simulink model "SEA_LQG_nonlinear"  (R2025b)
settings: Solver=ode23t  StartTime=0.0  StopTime=4  MaxStep=0.0050000000000000001  RelTol=1.0000000000000001e-05  AbsTol=9.9999999999999995e-08
Description:
  | explicit LQR plus Kalman observer -> M3 actuators -> nonlinear M1 SEA
settings Model: Creator=aless  LastModifiedBy=aless

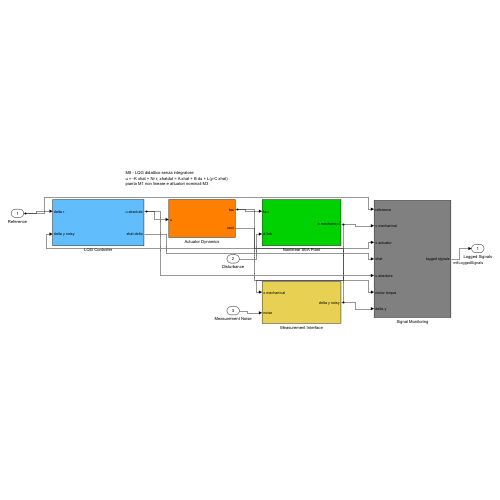
[thumbnail: Simulink's stored preview of the top-level diagram]
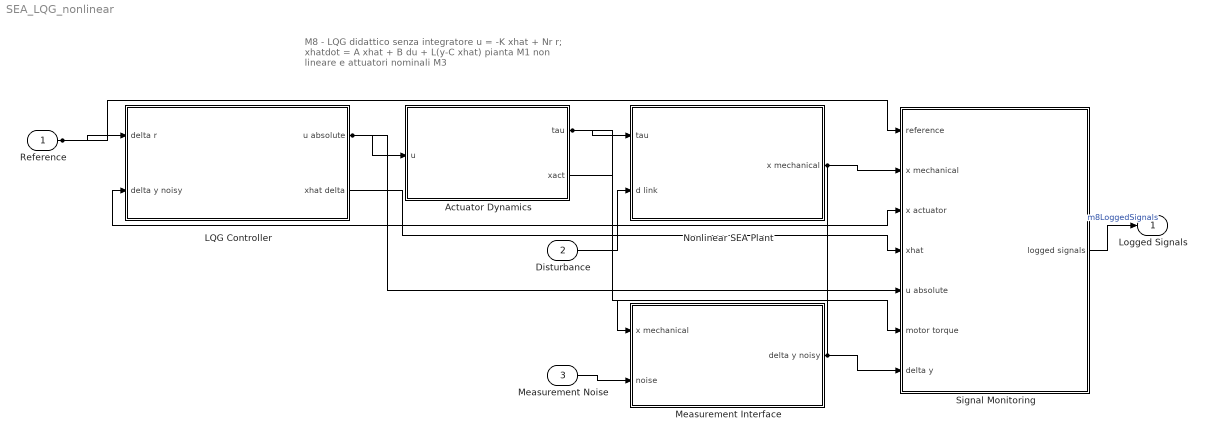
== system SEA_LQG_nonlinear ==
  note: M8 - LQG didattico senza integratore
      | u = -K xhat + Nr r; xhatdot = A xhat + B du + L(y-C xhat)
      | pianta M1 non lineare e attuatori nominali M3
  Reference : Inport  PortDimensions=2
  Disturbance : Inport  Port=2  PortDimensions=2
  Measurement Noise : Inport  Port=3  PortDimensions=4
  Actuator Dynamics : Subsystem
  LQG Controller : Subsystem
  Measurement Interface : Subsystem
  Nonlinear SEA Plant : Subsystem
  Signal Monitoring : Subsystem
  Logged Signals : Outport
  wires:
  Reference/1 -> LQG Controller/1(delta r), Signal Monitoring/1(reference)
  Measurement Interface/1(delta y noisy) -> LQG Controller/2(delta y noisy), Signal Monitoring/7(delta y)
  LQG Controller/1(u absolute) -> Actuator Dynamics/1(u), Signal Monitoring/5(u absolute)
  Actuator Dynamics/1(tau) -> Nonlinear SEA Plant/1(tau), Signal Monitoring/6(motor torque)
  Disturbance/1 -> Nonlinear SEA Plant/2(d link)
  Nonlinear SEA Plant/1(x mechanical) -> Measurement Interface/1(x mechanical), Signal Monitoring/2(x mechanical)
  Measurement Noise/1 -> Measurement Interface/2(noise)
  Actuator Dynamics/2(xact) -> Signal Monitoring/3(x actuator)
  LQG Controller/2(xhat delta) -> Signal Monitoring/4(xhat)
  Signal Monitoring/1(logged signals) -> Logged Signals/1  "m8LoggedSignals"

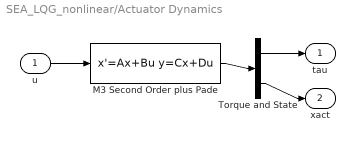
== system SEA_LQG_nonlinear/Actuator Dynamics ==
  u : Inport  PortDimensions=2
  M3 Second Order plus Pade : StateSpace  A=[-197.33333333333334 -79.166666666666671 -52.083333333333336 0 0 0;128 0 0 0 0 0;0 32 0 0 0 0;0 0 0 -197.33333333333334 -79.166666666666671 -52.083333333333336;0 0 0 128 0 0;0 0 0 0 32 0]  B=[8 0;0 0;0 0;0 8;0 0;0 0]  C=[0 -1.5625 6.510416666666667 0 0 0;0 0 0 0 -1.5625 6.510416666666667;1 0 0 0 0 0;0 1 0 0 0 0;0 0 1 0 0 0;0 0 0 1 0 0;0 0 0 0 1 0;0 0 0 0 0 1]  D=[0 0;0 0;0 0;0 0;0 0;0 0;0 0;0 0]  InitialCondition=[0;0;8.8575234782592865e-17;0;0;2.2143808695648216e-17]
  Torque and State : Demux  Outputs=[2 6]
  tau : Outport
  xact : Outport  Port=2
  wires:
  u/1 -> M3 Second Order plus Pade/1
  M3 Second Order plus Pade/1 -> Torque and State/1
  Torque and State/1 -> tau/1
  Torque and State/2 -> xact/1

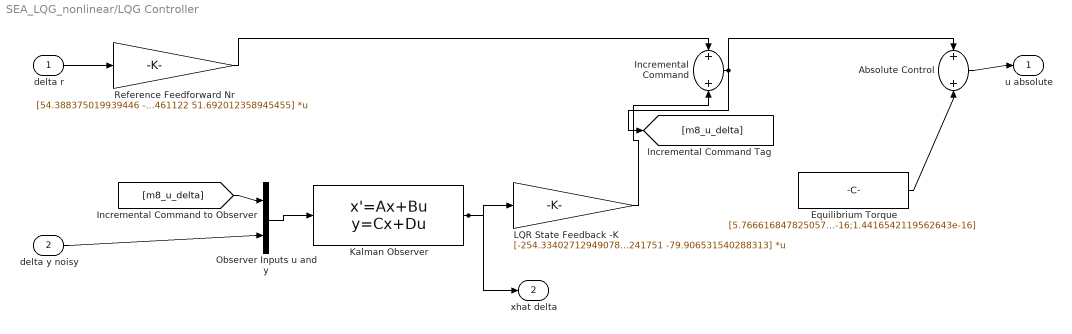
== system SEA_LQG_nonlinear/LQG Controller ==
  delta r : Inport  PortDimensions=2
  delta y noisy : Inport  Port=2  PortDimensions=4
  Absolute Control : Sum
  Equilibrium Torque : Constant  Value=[5.766616847825057e-16;1.4416542119562643e-16]
  Incremental Command : Sum
  Kalman Observer : StateSpace  A=[-22.708602708322911 21.793600911689683 1 0 -9.0440803445696254 5.5226633937677452 0 0 0 0 0 0 0 0;21.793600911690966 -85.604320358251826 0 1 6.9226259293456325 -23.470979906457924 0 0 0 0 0 0 0 0;-839.44343895121312 1838.0863088093163 0 0 79.231545442824768 -233.95675516648708 0 0 0 0 0 0 0 0;1983.0284167279717 -6039.1218427782769 0 0 -347.56991299100787 706.11322932558824 0 0 0 0 0 0 0 0;-9.0440803445693483 6.9226259293442176 0 0 -64.379631998469478 3.421864338890741 1 0 0 0 0 0 0 0;5.5226633937682017 -23.470979906457945 0 0 3.4218643388915506 -79.196108971786572 0 1 0 0 0 0 0 0;4275.8687111143208 934.10363067824846 0 0 -7143.0821554243939 313.4488480155174 -2 0 0 -156.25 651.04166666666674 0 0 0;755.87362777812768 1198.4788631876099 0 0 390.2760854773058 -7432.5597702775658 0 -2 0 0 0 0 -156.25 651.04166666666674;0.41526297627126696 2.254054873951131 0 0 35.114552541148264 1.7286492797991677 0 0 -197.33333333333334 -79.166666666666671 -52.083333333333336 0 0 0;-24.319927449188871 -14.409023934576732 0 0 92.13651423381539 0.28862886679991817 0 0 128 0 0 0 0 0;30.066433915707986 12.673170158948555 0 0 -207.8279927246254 -4.7947871057936995 0 0 0 32 0 0 0 0;1.9578954483030317 -4.8132582922373981 0 0 1.7024879035052436 30.031818202917915 0 0 0 0 0 -197.33333333333334 -79.166666666666671 -52.083333333333336;-11.539925704793928 9.1650966677943853 0 0 -1.3604732519714573 101.985096573353 0 0 0 0 0 128 0 0;9.7588925544826317 0.59061749336000824 0 0 -2.6169632704474655 -207.4223782133657 0 0 0 0 0 0 32 0]  B=[0 0 22.708602708322911 -21.793600911689683 9.0440803445696254 -5.5226633937677452;0 0 -21.793600911690966 85.604320358251826 -6.9226259293456325 23.470979906457924;0 0 551.4684389512131 -1274.3729754759829 233.26845455717523 -349.37657816684629;0 0 -1278.3867500613051 4200.9351761116104 -381.59675367565876 1210.5534373410785;0 0 9.0440803445693483 -6.9226259293442176 64.379631998469478 -3.421864338890741;0 0 -5.5226633937682017 23.470979906457945 -3.4218643388915506 79.196108971786572;0 0 724.13128888567894 -934.10363067824846 2143.0821554243939 -313.4488480155174;0 0 -755.87362777812768 2801.5211368123901 -390.2760854773058 3432.5597702775658;8 0 -0.41526297627126696 -2.254054873951131 -35.114552541148264 -1.7286492797991677;0 0 24.319927449188871 14.409023934576732 -92.13651423381539 -0.28862886679991817;0 0 -30.066433915707986 -12.673170158948555 207.8279927246254 4.7947871057936995;0 8 -1.9578954483030317 4.8132582922373981 -1.7024879035052436 -30.031818202917915;0 0 11.539925704793928 -9.1650966677943853 1.3604732519714573 -101.985096573353;0 0 -9.7588925544826317 -0.59061749336000824 2.6169632704474655 207.4223782133657]  C=[1 0 0 0 0 0 0 0 0 0 0 0 0 0;0 1 0 0 0 0 0 0 0 0 0 0 0 0;0 0 1 0 0 0 0 0 0 0 0 0 0 0;0 0 0 1 0 0 0 0 0 0 0 0 0 0;0 0 0 0 1 0 0 0 0 0 0 0 0 0;0 0 0 0 0 1 0 0 0 0 0 0 0 0;0 0 0 0 0 0 1 0 0 0 0 0 0 0;0 0 0 0 0 0 0 1 0 0 0 0 0 0;0 0 0 0 0 0 0 0 1 0 0 0 0 0;0 0 0 0 0 0 0 0 0 1 0 0 0 0;0 0 0 0 0 0 0 0 0 0 1 0 0 0;0 0 0 0 0 0 0 0 0 0 0 1 0 0;0 0 0 0 0 0 0 0 0 0 0 0 1 0;0 0 0 0 0 0 0 0 0 0 0 0 0 1]  D=[0 0 0 0 0 0;0 0 0 0 0 0;0 0 0 0 0 0;0 0 0 0 0 0;0 0 0 0 0 0;0 0 0 0 0 0;0 0 0 0 0 0;0 0 0 0 0 0;0 0 0 0 0 0;0 0 0 0 0 0;0 0 0 0 0 0;0 0 0 0 0 0;0 0 0 0 0 0;0 0 0 0 0 0]  InitialCondition=[0;0;0;0;0;0;0;0;0;0;0;0;0;0]
  LQR State Feedback -K : Gain  Gain=[-254.33402712949078 -15.858170528922438 -18.863074097404091 -3.8087455961462471 166.28258478745431 12.948051636244728 1.2986315941528244 0.91762390858549392 -11.555087565124021 -22.016226347778417 -42.310051575647563 0.97375969577285126 2.3551817304053437 13.48339013278521;-14.930135066522146 -213.75368485866457 -4.6969249142302845 -7.3299167336066668 5.5369618131759939 143.45950296172026 0.64525993536726456 -1.3209293150875645 0.97375969577245258 2.2226645703274865 10.907506609063152 -14.330897717523571 -28.541055981241751 -79.906531540288313]  Multiplication=Matrix(K*u)
  Observer Inputs u and y : Mux  Inputs=2
  Reference Feedforward Nr : Gain  Gain=[54.388375019939446 -1.2769983608264373;3.4068130335461122 51.692012358945455]  Multiplication=Matrix(K*u)
  u absolute : Outport
  xhat delta : Outport  Port=2
  wires:
  delta r/1 -> Reference Feedforward Nr/1
  Reference Feedforward Nr/1 -> Incremental Command/1
  Kalman Observer/1 -> LQR State Feedback -K/1, xhat delta/1
  LQR State Feedback -K/1 -> Incremental Command/2
  Incremental Command/1 -> [m8_u_delta], Absolute Control/1
  [m8_u_delta] -> Observer Inputs u and y/1
  delta y noisy/1 -> Observer Inputs u and y/2
  Observer Inputs u and y/1 -> Kalman Observer/1
  Equilibrium Torque/1 -> Absolute Control/2
  Absolute Control/1 -> u absolute/1

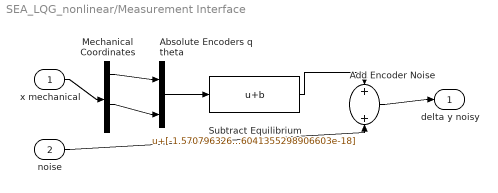
== system SEA_LQG_nonlinear/Measurement Interface ==
  x mechanical : Inport  PortDimensions=8
  noise : Inport  Port=2  PortDimensions=4
  Absolute Encoders q theta : Mux  Inputs=2
  Add Encoder Noise : Sum
  Mechanical Coordinates : Demux  Outputs=[2 2 2 2]
  Subtract Equilibrium : Bias  Bias=[-1.5707963267948966;0;-1.5707963267948966;-3.6041355298906603e-18]  SaturateOnIntegerOverflow=off
  delta y noisy : Outport
  wires:
  x mechanical/1 -> Mechanical Coordinates/1
  Mechanical Coordinates/1 -> Absolute Encoders q theta/1
  Mechanical Coordinates/3 -> Absolute Encoders q theta/2
  Absolute Encoders q theta/1 -> Subtract Equilibrium/1
  Subtract Equilibrium/1 -> Add Encoder Noise/1
  noise/1 -> Add Encoder Noise/2
  Add Encoder Noise/1 -> delta y noisy/1

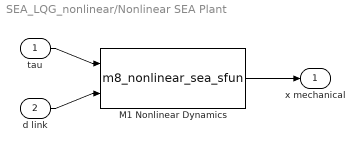
== system SEA_LQG_nonlinear/Nonlinear SEA Plant ==
  tau : Inport  PortDimensions=2
  d link : Inport  Port=2  PortDimensions=2
  M1 Nonlinear Dynamics : M-S-Function  FunctionName=m8_nonlinear_sea_sfun  Parameters=[1.5707963267948966;0;0;0;1.5707963267948966;3.6041355298906603e-18;0;0]
  x mechanical : Outport
  wires:
  tau/1 -> M1 Nonlinear Dynamics/1
  d link/1 -> M1 Nonlinear Dynamics/2
  M1 Nonlinear Dynamics/1 -> x mechanical/1

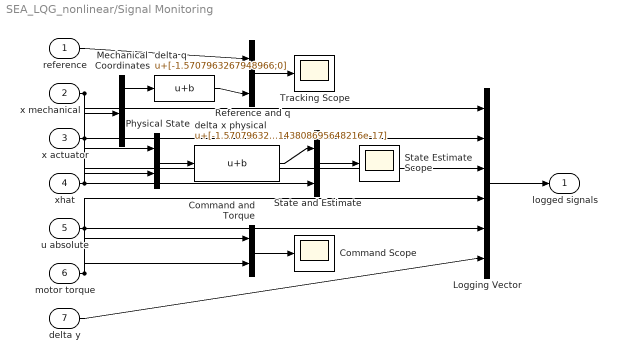
== system SEA_LQG_nonlinear/Signal Monitoring ==
  reference : Inport  PortDimensions=2
  x mechanical : Inport  Port=2  PortDimensions=8
  x actuator : Inport  Port=3  PortDimensions=6
  xhat : Inport  Port=4  PortDimensions=14
  u absolute : Inport  Port=5  PortDimensions=2
  motor torque : Inport  Port=6  PortDimensions=2
  delta y : Inport  Port=7  PortDimensions=4
  Command Scope : Scope
  Command and Torque : Mux  Inputs=2
  Logging Vector : Mux  Inputs=6
  Mechanical Coordinates : Demux  Outputs=[2 2 2 2]
  Physical State : Mux  Inputs=2
  Reference and q : Mux  Inputs=2
  State Estimate Scope : Scope
  State and Estimate : Mux  Inputs=2
  Tracking Scope : Scope
  delta q : Bias  Bias=[-1.5707963267948966;0]  SaturateOnIntegerOverflow=off
  delta x physical : Bias  Bias=[-1.5707963267948966;0;0;0;-1.5707963267948966;-3.6041355298906603e-18;0;0;0;0;-8.8575234782592865e-17;0;0;-2.2143808695648216e-17]  SaturateOnIntegerOverflow=off
  logged signals : Outport
  wires:
  x mechanical/1 -> Mechanical Coordinates/1, Physical State/1, Logging Vector/1
  reference/1 -> Reference and q/1
  Mechanical Coordinates/1 -> delta q/1
  delta q/1 -> Reference and q/2
  Reference and q/1 -> Tracking Scope/1
  x actuator/1 -> Physical State/2, Logging Vector/2
  Physical State/1 -> delta x physical/1
  delta x physical/1 -> State and Estimate/1
  xhat/1 -> State and Estimate/2, Logging Vector/3
  State and Estimate/1 -> State Estimate Scope/1
  u absolute/1 -> Command and Torque/1, Logging Vector/4
  motor torque/1 -> Command and Torque/2, Logging Vector/5
  Command and Torque/1 -> Command Scope/1
  delta y/1 -> Logging Vector/6
  Logging Vector/1 -> logged signals/1
